simulink model "model_tp2"  (R2024a)
settings: Solver=VariableStepAuto  StartTime=0.0  StopTime=200  RelTol=1e-3
InitFcn:
  | initdata
values from neighbouring files (symbols this model uses):
  K = place(A_mimo,B_mimo,lambda_spec)    [initdata.m]    (also in mainv2.m = convhulln(x_opt'); mainv3.m = convhulln(x_opt'); mainv4.m = convhulln(x_opt'); mainv5.m = convhulln(x_opt'))
undefined symbols (not defined in the file or in its folder): A_int, B_int, C_int, D_int, Kn
settings Model: Creator=paulogil  LastModifiedBy=Utilizador
settings SolverCC: AlgebraicLoopSolver=TrustRegion
settings DebuggingCC: UnconnectedInputMsg=warning  UnconnectedOutputMsg=warning  UnconnectedLineMsg=warning  ArithmeticOperatorsInVariantConditions=warning
settings ModelReferenceCC: EnableRefExpFcnMdlSchedulingChecks=on
settings SFSimCC: CustomCodeUndefinedFunction=UseInterfaceOnly
settings RTWCC: GPUComputeCapability=3.5

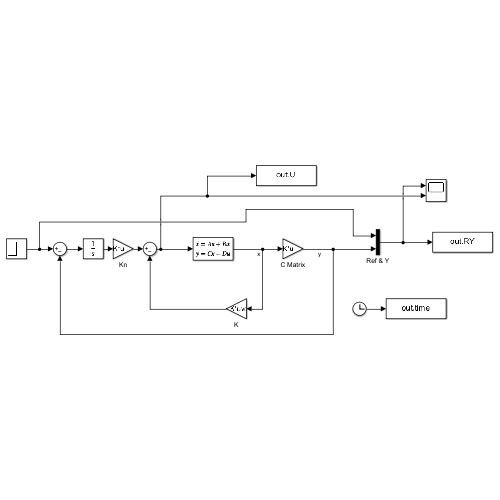
[thumbnail: Simulink's stored preview of the top-level diagram]
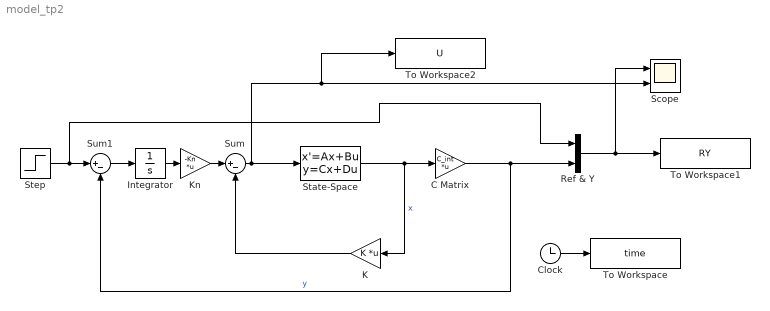
== system model_tp2 ==
  C Matrix : Gain  Gain=C_int  Multiplication=Matrix(K*u)
  Clock : Clock
  Integrator : Integrator
  K : Gain  Gain=K  Multiplication=Matrix(K*u) (u vector)
  Kn : Gain  Gain=-Kn  Multiplication=Matrix(K*u)
  Ref & Y : Mux  Inputs=2
  Scope : Scope  NumInputPorts=2
  State-Space : StateSpace  A=A_int  B=B_int  C=C_int  D=D_int  InitialCondition=0
  Step : Step  Time=0  After=0.5  SampleTime=0
  Sum : Sum  Inputs=|+-
  Sum1 : Sum  Inputs=|+-
  To Workspace : ToWorkspace  VariableName=time  SaveFormat=Timeseries  SampleTime=-1
  To Workspace1 : ToWorkspace  VariableName=RY  SaveFormat=Timeseries  SampleTime=-1
  To Workspace2 : ToWorkspace  VariableName=U  SaveFormat=Timeseries  SampleTime=-1
  wires:
  K/1 -> Sum/2
  Integrator/1 -> Kn/1
  Step/1 -> Sum1/1, Ref & Y/1
  C Matrix/1 -> Sum1/2, Ref & Y/2  "y"
  Ref & Y/1 -> To Workspace1/1, Scope/1
  Clock/1 -> To Workspace/1
  Sum1/1 -> Integrator/1
  Kn/1 -> Sum/1
  State-Space/1 -> C Matrix/1, K/1  "x"
  Sum/1 -> State-Space/1, To Workspace2/1, Scope/2
